simulink model "gm_PMLSM_FOC_FixedPoint"  (R2026b)
settings: Solver=FixedStepDiscrete  StopTime=.01  FixedStep=2e-08
undefined symbols (not defined in the file): Lookup, Ts_ACR
libraries: hdlmdlgenlib x38, simulink x8
(part 3 of 5)

== system gm_PMLSM_FOC_FixedPoint/FOC_DUT/FOC_DUT/InversePark/Variant/mcb/sinecos/Sine-Cosine Lookup ==
  Theta : Inport  OutDataTypeStr=fixdt(1, 40, 32)  PortDimensions=1  SampleTime=0.0001
  Data Type Conversion1 : DataTypeConversion  OutDataTypeStr=fixdt(1, 40, 29)  RndMeth=Simplest  SampleTime=0.0001  SaturateOnIntegerOverflow=off
  Get_Integer : DataTypeConversion  OutDataTypeStr=uint16  RndMeth=Simplest  SampleTime=0.0001  SaturateOnIntegerOverflow=off
  Interpolation : Subsystem
  Lookup : Selector  IndexMode=Zero-based  InputPortWidth=1002  IndexOptions=Index vector (port)  Indices=double([1 3])  OutputSizes=1
  Sum : Sum  OutDataTypeStr=uint32  AccumDataTypeStr=uint32  RndMeth=Simplest  SampleTime=0.0001
  Sum2 : Sum  Inputs=+-  OutDataTypeStr=fixdt(1, 40, 32)  AccumDataTypeStr=fixdt(1, 40, 29)  RndMeth=Simplest  SampleTime=0.0001
  WrapUp : Subsystem
  datatype : Subsystem
  indexing : Gain  Gain="fi(0,1,40,29,\"hex\",\"6400000000\")"  ParamDataTypeStr=fixdt(1, 40, 29)  OutDataTypeStr=fixdt(1, 80, 61)  SampleTime=0.0001
  indexing_out_dtc : DataTypeConversion  OutDataTypeStr=fixdt(1, 40, 29)  RndMeth=Simplest  SampleTime=0.0001  SaturateOnIntegerOverflow=off
  offset : Constant  Value=[1;0;201;200]  OutDataTypeStr=int16  SampleTime=0.0001
  sine_table_values : Constant  Value=[0;0.00785390078090131282806396484375;0.0157073172740638256072998046875;0.02355976472608745098114013671875;0.03141075908206403255462646484375;0.03925981582142412662506103515625;0.04710645065642893314361572265625;0.0549501799978315830230712890625;0.062790519557893276214599609375;0.07062698598019778728485107421875;0.0784590956754982471466064453125;0.08628636575303971767425537109375;0.0941083133220672607421875;0.101924455724656581878662109375;0.10973431100137531757354736328125;0.1175373974256217479705810546875;0.12533323350362479686737060546875;0.13312133844010531902313232421875;0.14090123190544545650482177734375;0.14867243380285799503326416015625;0.15643446496687829494476318359375;0.1641868464648723602294921875;0.17192910029552876949310302734375;0.1796607486903667449951171875;0.1873813145793974399566650390625;0.19509032205678522586822509765625;0.2027872954495251178741455078125;0.21047175978310406208038330078125;0.21814324147999286651611328125;0.22580126696266233921051025390625;0.23344536381773650646209716796875;0.2410750607959926128387451171875;0.248689887113869190216064453125;0.256289373151957988739013671875;0.26387304998934268951416015625;0.27144044986926019191741943359375;0.278991105966269969940185546875;0.28652455261908471584320068359375;0.29404032533057034015655517578125;0.301537959836423397064208984375;0.30901699443347752094268798828125;0.3164769671857357025146484375;0.3239174182526767253875732421875;0.33133788849227130413055419921875;0.33873792015947401523590087890625;0.34611705713905394077301025390625;0.3534748437814414501190185546875;0.360810826532542705535888671875;0.36812455276958644390106201171875;0.37541557126678526401519775390625;0.38268343242816627025604248046875;0.38992768782190978527069091796875;0.3971478906460106372833251953125;0.40434359549544751644134521484375;0.41151435859501361846923828125;0.41865973756648600101470947265625;0.42577929166145622730255126953125;0.43287258152849972248077392578125;0.43993916991166770458221435546875;0.4469786207191646099090576171875;0.45399049972184002399444580078125;0.46097437455318868160247802734375;0.46792981424368917942047119140625;0.47485638991929590702056884765625;0.48175367410294711589813232421875;0.488621241413056850433349609375;0.49545866833068430423736572265625;0.50226553319953382015228271484375;0.50904141576029360294342041015625;0.51578589831478893756866455078125;0.52249856479465961456298828125;0.52917900099419057369232177734375;0.53582679503597319126129150390625;0.542441536672413349151611328125;0.54902281798422336578369140625;0.55557023291476070880889892578125;0.5620833779685199260711669921875;0.56856185081414878368377685546875;0.57500525214709341526031494140625;0.581413184292614459991455078125;0.587785252369940280914306640625;0.59412106289528310298919677734375;0.6004202254116535186767578125;0.60668235109187662601470947265625;0.61290705366991460323333740234375;0.61909394920803606510162353515625;0.62524265632964670658111572265625;0.63135279552079737186431884765625;0.6374239898286759853363037109375;0.64345586462877690792083740234375;0.6494480483233928680419921875;0.655400170944631099700927734375;0.6613118653185665607452392578125;0.667182766832411289215087890625;0.67301251343451440334320068359375;0.67880074563436210155487060546875;0.68454710603691637516021728515625;0.69025124027393758296966552734375;0.6959127965383231639862060546875;0.70153142581693828105926513671875;0.707106781192123889923095703125;0.71263851900584995746612548828125;0.71812629769556224346160888671875;0.7235697791911661624908447265625;0.72896862751804292201995849609375;0.73432250949554145336151123046875;0.739631094969809055328369140625;0.744894056580960750579833984375;0.7501110695302486419677734375;0.75528181227855384349822998046875;0.7604059656150639057159423828125;0.76548321358859539031982421875;0.77051324280910193920135498046875;0.77549574314616620540618896484375;0.780430407263338565826416015625;0.78531693085096776485443115234375;0.79015501239337027072906494140625;0.794944353401660919189453125 ...(+30284 chars)]  OutDataTypeStr=fixdt(1, 40, 32)  SampleTime=0.0001
  sin : Outport  OutDataTypeStr=fixdt(1, 40, 32)  PortDimensions=1  SampleTime=0.0001  VectorParamsAs1DForOutWhenUnconnected=off
  cos : Outport  Port=2  OutDataTypeStr=fixdt(1, 40, 32)  PortDimensions=1  SampleTime=0.0001  VectorParamsAs1DForOutWhenUnconnected=off
  wires:
  Interpolation/1(Out1) -> sin/1
  indexing_out_dtc/1 -> Sum2/1, Get_Integer/1
  Theta/1 -> WrapUp/1(In1)
  sine_table_values/1 -> Lookup/1
  Get_Integer/1 -> Data Type Conversion1/1, Sum/1
  WrapUp/1(Out1) -> indexing/1
  indexing/1 -> indexing_out_dtc/1
  offset/1 -> Sum/2
  Sum/1 -> Lookup/2
  Data Type Conversion1/1 -> Sum2/2
  Lookup/1 -> datatype/1(In1)
  Sum2/1 -> Interpolation/2(In2)
  datatype/1(Out1) -> Interpolation/1(In1)
  Interpolation/2(Out2) -> cos/1

== system gm_PMLSM_FOC_FixedPoint/FOC_DUT/FOC_DUT/Park/Variant/mcb/Park Transform/Select ==
  AlphaIn : Inport  OutDataTypeStr=fixdt(1, 64, 40)  PortDimensions=1  SampleTime=2e-08
  BetaIn : Inport  Port=2  OutDataTypeStr=fixdt(1, 64, 40)  PortDimensions=1  SampleTime=2e-08
  Sin : Inport  Port=3  OutDataTypeStr=fixdt(1, 40, 32)  PortDimensions=1  SampleTime=2e-08
  Cos : Inport  Port=4  OutDataTypeStr=fixdt(1, 40, 32)  PortDimensions=1  SampleTime=2e-08
  Two Inputs : Subsystem
  D : Outport  OutDataTypeStr=fixdt(1, 64, 40)  PortDimensions=1  SampleTime=2e-08  VectorParamsAs1DForOutWhenUnconnected=off
  Q : Outport  Port=2  OutDataTypeStr=fixdt(1, 64, 40)  PortDimensions=1  SampleTime=2e-08
  wires:
  Two Inputs/1(D) -> D/1
  AlphaIn/1 -> Two Inputs/1(AlphaIn)
  Two Inputs/2(Q) -> Q/1
  BetaIn/1 -> Two Inputs/2(BetaIn)
  Sin/1 -> Two Inputs/3(Sin)
  Cos/1 -> Two Inputs/4(Cos)
